simulink model "PID"  (R2026a)
settings: Solver=VariableStepAuto  StopTime=10
values from neighbouring files (symbols this model uses):
  Ad = expm(A*Ts)    [paramEncomendadoc.m]
  Bd = integral(@(t) expm(A*t)*B,0,Ts,'ArrayValued',true)    [paramEncomendadoc.m]
  PID_Kd = -12    [paramEncomendadoc.m]
  PID_Ki = 0    [paramEncomendadoc.m]
  PID_Kp = -109    [paramEncomendadoc.m]
  PID_Kw = -0.47    [paramEncomendadoc.m]
  Ts = 0.001    [paramEncomendadoc.m]
  x0 = [deg2rad(10); 0; 0]    [paramEncomendadoc.m]
libraries: slpidlib x1
settings Model: Creator=Agmar  LastModifiedBy=Enzo

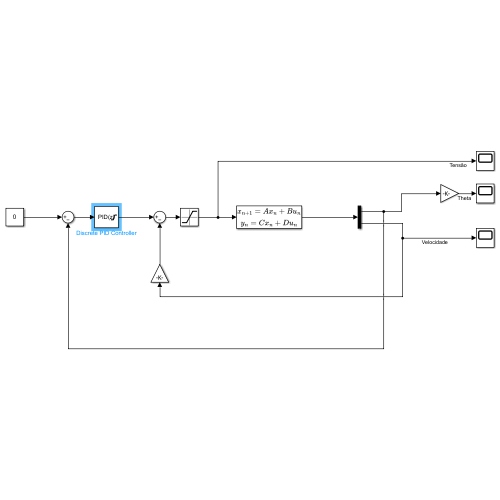
[thumbnail: Simulink's stored preview of the top-level diagram]
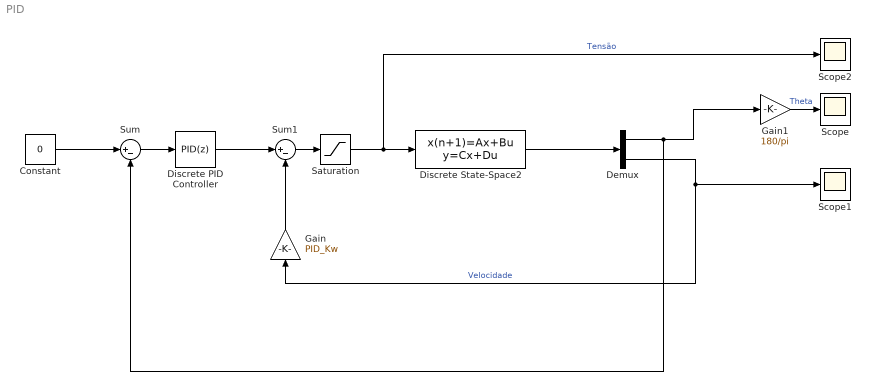
== system PID ==
  Constant : Constant  Value=0  SampleTime=Ts
  Demux : Demux  Outputs=2
  Discrete PID Controller : slpidlib/PID Controller  Controller=PID  Form=Parallel  TimeDomain=Discrete-time  UseExternalTs=off  SampleTime=Ts  IntegratorMethod=Trapezoidal  FilterMethod=Trapezoidal  ControllerParametersSource=internal  P=PID_Kp  I=PID_Ki  UseKiTs=off  D=PID_Kd  UseExternalDerivativeSource=off  N=100  UseFilter=on  TunerSelectOption=Transfer Function Based (PID Tuner App)  InitialConditionSource=internal  InitialConditionForIntegrator=0  InitialConditionForFilter=0  DifferentiatorICPrevScaledInput=0  ExternalReset=none  TrackingMode=off  Kt=1  LimitOutput=on  SatLimitsSource=internal  UpperSaturationLimit=18  LowerSaturationLimit=-18  LinearizeAsGain=off  AntiWindupMode=clamping  Kb=1  LimitIntegrator=off  UpperIntegratorSaturationLimit=inf  LowerIntegratorSaturationLimit=-inf  POutMin=[]  POutMax=[]  IOutMin=[]  IOutMax=[]  DOutMin=[]  DOutMax=[]  NOutMin=[]  NOutMax=[]  SumOutMin=[]  SumOutMax=[]  SaturationOutMin=[]  SaturationOutMax=[]  PParamMin=[]  PParamMax=[]  IParamMin=[]  IParamMax=[]  DParamMin=[]  DParamMax=[]  NParamMin=[]  NParamMax=[]  KbParamMin=[]  KbParamMax=[]  KtParamMin=[]  KtParamMax=[]  KbOutMin=[]  KbOutMax=[]  KtOutMin=[]  KtOutMax=[]  IntegratorOutMin=[]  IntegratorOutMax=[]  FilterOutMin=[]  FilterOutMax=[]  SumI1OutMin=[]  SumI1OutMax=[]  SumI2OutMin=[]  SumI2OutMax=[]  SumI3OutMin=[]  SumI3OutMax=[]  SumI4OutMin=[]  SumI4OutMax=[]  SumDOutMin=[]  SumDOutMax=[]  DifferentiatorOutMin=[]  DifferentiatorOutMax=[]  FilterDiffOutCoefMin=[]  FilterDiffOutCoefMax=[]  ReciprocalOutMin=[]  ReciprocalOutMax=[]  SumDenOutMin=[]  SumDenOutMax=[]  SumNumOutMin=[]  SumNumOutMax=[]  DivideOutMin=[]  DivideOutMax=[]  UdiffTsProdOutMin=[]  UdiffTsProdOutMax=[]  NTsProdOutMin=[]  NTsProdOutMax=[]  UintegralTsProdOutMin=[]  UintegralTsProdOutMax=[]  UngainTsProdOutMin=[]  UngainTsProdOutMax=[]  ClampingZeroOutDataTypeStr=Inherit: Inherit via back propagation  ClampingZeroOutMin=[]  ClampingZeroOutMax=[]  FilterDenConstantOutDataTypeStr=Inherit: Inherit via back propagation  FilterDenConstantOutMin=[]  FilterDenConstantOutMax=[]  PCopyOutDataTypeStr=Inherit: Inherit via back propagation  PCopyOutMin=[]  PCopyOutMax=[]  NCopyOutDataTypeStr=Inherit: Inherit via back propagation  NCopyOutMin=[]  NCopyOutMax=[]  IntegratorContinuousStateAttributes=''  IntegratorStateMustResolveToSignalObject=off  IntegratorRTWStateStorageClass=Auto  FilterContinuousStateAttributes=''  FilterStateMustResolveToSignalObject=off  FilterRTWStateStorageClass=Auto  ParallelPVariant=InternalParameters  IdealPVariant=Disabled  IVariant=InternalParameters  DVariant=InternalParameters  IntegratorVariant=Discrete  SatVariant=Enabled  AWVariant=DiscClampingParallel  PCopyVariant=Disabled  TRVariant=Disabled  FdbkBlocksVariant=Feedback  IdealPFdbkVariant=Passthrough  SatFdbkVariant=Passthrough  DerivativeFilterVariant=TrapezoidalFilter  NVariant=InternalParameters  NCopyVariant=InternalParameters  FilterICVariant=InternalICsFilter  IntegratorICVariant=InternalICs  ExternalResetVariant=Disabled  TRSumVariant=Passthrough  SumFdbkVariant=Enabled  SumVariant=Sum_PID  TsampFilterVariant=InternalTs  TsampNgainVariant=Passthrough  TsampIntegralVariant=Disabled_SignalSpec  ExternalSaturationOutDataTypeStr=Inherit: Same as second input  DerivativeSourceVariant=ErrorSignal  PreIntVariant=InternalPreInt
      settings: LibrarySourceBlock=simulink/Discrete/Discrete PID Controller
  Discrete State-Space2 : DiscreteStateSpace  A=Ad  B=Bd  C=[1 0 0; 0 0 1]  D=[0; 0]  InitialCondition=x0  SampleTime=Ts
  Gain : Gain  Gain=PID_Kw
  Gain1 : Gain  Gain=180/pi
  Saturation : Saturate  UpperLimit=18  LowerLimit=-18
  Scope : Scope
      settings: ActiveDisplayYMinimum=-3.714543802676082  ActiveDisplayYMaximum=11.523838200297343
  Scope1 : Scope
      settings: ActiveDisplayYMinimum=-2.2375983676583506  ActiveDisplayYMaximum=20.138385308925159
  Scope2 : Scope
      settings: ActiveDisplayYMinimum=-2.2601610427093353  ActiveDisplayYMaximum=20.251129004745483  DataLoggingVariableName=ScopeData2
  Sum : Sum  Inputs=|+-
  Sum1 : Sum  Inputs=|+-
  wires:
  Constant/1 -> Sum/1
  Sum1/1 -> Saturation/1
  Gain/1 -> Sum1/2
  Sum/1 -> Discrete PID Controller/1
  Discrete PID Controller/1 -> Sum1/1
  Saturation/1 -> Discrete State-Space2/1, Scope2/1  "Tensão"
  Gain1/1 -> Scope/1  "Theta"
  Discrete State-Space2/1 -> Demux/1
  Demux/1 -> Sum/2, Gain1/1
  Demux/2 -> Gain/1, Scope1/1  "Velocidade"
